simulink model "DEMOIO"  (Simulink 7.0)
settings: Solver=FixedStepDiscrete  StartTime=0.0  StopTime=10  FixedStep=0.0001  RelTol=1e-3
undefined symbols (not defined in the file or in its folder): OC1max
libraries: dsPICdrivers x4
CloseFcn:
  | rtwprivate ssgencode ModelCloseRequest speed_current_control
settings Model: Creator=Lubin  LastModifiedBy=MATLABMICROCHIP
settings SolverCC: PositivePriorityOrder=on  AutoInsertRateTranBlk=on
settings DataIOCC: Decimation=4  MaxDataPoints=65536
settings OptimizationCC: OptimizeModelRefInitCode=on  LifeSpan=1
settings DebuggingCC: SaveWithParameterizedLinksMsg=none  SignalResolutionControl=TryResolveAllWithWarning
settings HardwareCC: ProdBitPerInt=16  ProdEndianess=LittleEndian  ProdWordSize=16  ProdHWDeviceType=16-bit Generic  TargetHWDeviceType=32-bit Generic
settings RTWCC: SystemTargetFile=dspic.tlc  TemplateMakefile=dspic_pic30_gcc.tmf  PostCodeGenCommand=dsPIC_Compile()  Description=Embedded Target for Microchip dsPIC (real-time)  ProcessScript=dspic_make_rtw_hook
settings CodeAppCC: IgnoreCustomStorageClasses=off
settings STFCustomTargetCC: GenFloatMathFcnCalls=ANSI_C  ModelReferenceCompliant=off  IncludeMdlTerminateFcn=off  CombineOutputUpdateFcns=on  SuppressErrorStatus=on  ERTCustomFileBanners=on  SupportContinuousTime=off  SupportNonInlinedSFcns=off  SystemTargetFile=dspic.tlc
settings ERTTargetCC: GenFloatMathFcnCalls=ANSI_C  ModelReferenceCompliant=off  CompOptLevelCompliant=off  IncludeMdlTerminateFcn=off  SuppressErrorStatus=on  ModelStepFunctionPrototypeControlCompliant=off  InlinedParameterPlacement=NonHierarchical  ERTSrcFileBannerTemplate=dsPIC_code_template.cgt  ERTHdrFileBannerTemplate=dsPIC_code_template.cgt  ERTDataSrcFileTemplate=dsPIC_code_template.cgt  ERTDataHdrFileTemplate=dsPIC_code_template.cgt  ERTCustomFileTemplate=dsPIC_main.tlc
settings CustomProperty: DataType=string  Value=C:\MATLAB~4\bin\win32\gmake

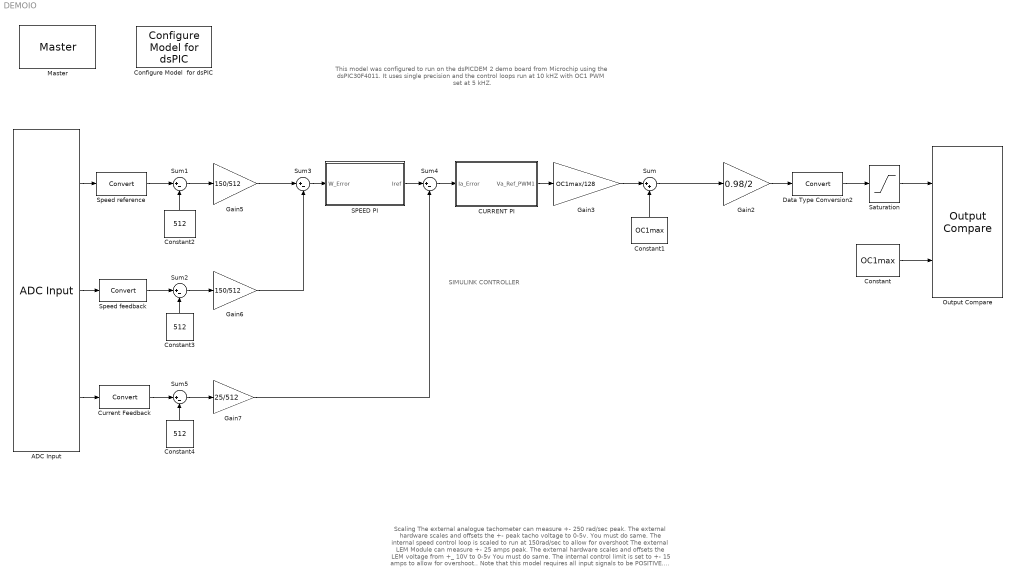
== system DEMOIO ==
  note: This model was configured to run on the dsPICDEM 2
      | demo board from Microchip using the  dsPIC30F4011.
      |
      | It uses single precision and the control loops run at 10 kHZ
      | with OC1 PWM set at  5 kHZ.
  note: Scaling
      |
      | The external analogue tachometer can measure +- 250 rad/sec peak. The external hardware scales and offsets the +- peak tacho voltage to  0-5v. You must do same. The internal speed control loop is scaled to run at 150rad/sec to allow for overshoot
      |
      | The external LEM Module can measure +- 25 amps peak. The external hardware scales and offsets the LEM voltage from +_ 10V to 0-5v You must do same. The internal control limit is set to +- 15 amps to allow for overshoot..
      |
      | Note that this model requires all input signals to be POSITIVE. The DC voltage is 128 volts. Change this to your desired output DC voltage.
      |
      | GOOD LUCK IT SHOULD WORK IF ALL THE FEEDBACK IS CORRECT.
      |
      | If you remove just the SIMULINK CNTROLLER you will be able to use the controllers in SIMULINK.
  note: SIMULINK CONTROLLER
  ADC Input : dsPICdrivers/Peripheral I//O/ADC Input  Tag=dsPIC_ADC  Priority=5  ADC_TYPE=10 bits  ADC_MODE=Continuous sampling & get last channel value  NbrSampleStep=1  VoltRefpopup="AVdd  -  AVss"  OutFormatBitspopup=0000 00dd dddd dddd : Integer  InterruptPriority=6  ANCHANNELS=[4 6 7]  MaxName=ANmax = 1024  Rin=1e2  ADCS=4  SAMC=1  Temperature=25  DMAChannel=0  SampleTime=0.0001  Status="OK  |  Tsmp=1.695e-007 |  T/Channel=2.204e-006 |  Tall=6.612e-006"
  CURRENT PI : Subsystem
  Configure Model  for dsPIC : dsPICdrivers/Simulink Configuration/Configure Model  for dsPIC
  Constant : Constant  Value=OC1max  OutDataTypeMode=uint16  OutDataType=sfix(16)  OutScaling=2^0  SampleTime=0.0001
  Constant1 : Constant  Orientation=up  Value=OC1max  OutDataTypeMode=single  OutDataType=sfix(16)  OutScaling=2^0  SampleTime=0.0001
  Constant2 : Constant  Orientation=up  Value=512  VectorParams1D=off  OutDataTypeMode=single  OutDataType=sfix(16)  OutScaling=2^0  SampleTime=0.0001
  Constant3 : Constant  Orientation=up  Value=512  OutDataTypeMode=single  OutDataType=sfix(16)  OutScaling=2^0  SampleTime=0.0001
  Constant4 : Constant  Orientation=up  Value=512  OutDataTypeMode=single  OutDataType=sfix(16)  OutScaling=2^0  SampleTime=0.0001
  Current Feedback : DataTypeConversion  OutDataTypeMode=single  OutDataType=sfix(16)  OutScaling=2^0  SampleTime=0.0001
  Data Type Conversion2 : DataTypeConversion  OutDataTypeMode=uint16  OutDataType=sfix(16)  OutScaling=2^0  SampleTime=0.0001
  Gain2 : Gain  Gain=0.98/2  ParameterDataType=sfix(16)  ParameterScaling=2^0  OutDataTypeMode=single  OutDataType=sfix(16)  OutScaling=2^0  SampleTime=0.0001
  Gain3 : Gain  Gain=OC1max/128  ParameterDataType=sfix(16)  ParameterScaling=2^0  OutDataTypeMode=single  OutDataType=sfix(16)  OutScaling=2^0  SampleTime=0.0001
  Gain5 : Gain  Gain=150/512  ParameterDataType=sfix(16)  ParameterScaling=2^0  OutDataType=sfix(16)  OutScaling=2^0  SampleTime=0.0001
  Gain6 : Gain  Gain=150/512  ParameterDataType=sfix(16)  ParameterScaling=2^0  OutDataType=sfix(16)  OutScaling=2^0  SampleTime=0.0001
  Gain7 : Gain  Gain=25/512  ParameterDataType=sfix(16)  ParameterScaling=2^0  OutDataType=sfix(16)  OutScaling=2^0  SampleTime=0.0001
  Master : dsPICdrivers/Master  Tag=dsPIC_MASTER  Priority=1  TimeStepType=Timer1  picType=30f4011  fcy=14745600  Quartz_33f=5e6  PLLActive_33f=off  fcyDesired_33f=0  tmr1="[1  1474  -0.029839]"  tmr1Info="Time Step : 0.00010003  ;   Error : -0.029839%  PR1=1474"  tmr2345="[1  0  0  0]"  tmr2345cfg=[-1 -1 -1 -1]  IOautoConf=on  typePort="[ 0  0  0  0  0  0  0  0  0  0  0  0  0  0  0  0  0  0  0  0  8  0  8  8  0  0  0  0  0  0  0  0  0  0  0  0  0  0  0  0  0  0  0  0  0  0  0  0  7  0  0  0  0  0  0  0  0  0  0  0  0  0  0  0  0  0  0  0  0  0  0  0  0  0  0  0  0  0  0  0  0  0  0  0  0  0  0  0  0  0  0  0  0  0  0  0  0  0  0  0  0  0  0  0  0  0  0  0  0  0  0  0 ]"  TRIS="[ 65535  65535  65535  65534  65535  65535  65535 ]"  ADPCFG=0  MasterBusyPort=None  MasterOverloadPort=None  FOSC=XT_PLL8  ClockSwitchMonitor=Both disabled  TempProtection_33f=TEMP_ON  FPBOR=PBOR_OFF  PWRT=PWRT_OFF  MCLR=MCLR_DIS  PowerSave=off  OverrideFcy=off  NewFcy=1e6
  Output Compare : dsPICdrivers/Peripheral I//O/Output Compare  Tag=dsPIC_PWM_out  Priority=5  IntPriority=3  CHANNEL=[1]  Channel_UP_Down_Periode=[5]  MaxChannel=[0.0002]  MaxName=' OC1max '  Precision=[11.5261]  Timer=[2]  Status=OK  SafeMarge=[0]  PortLetter=[68]  PortNumber=[0]  MaxValues=[2949.12]
  SPEED PI : Subsystem
  Saturation : Saturate  UpperLimit=OC1max  LowerLimit=0
  Speed feedback : DataTypeConversion  OutDataTypeMode=single  OutDataType=sfix(16)  OutScaling=2^0  SampleTime=0.0001
  Speed reference : DataTypeConversion  OutDataTypeMode=single  OutDataType=sfix(16)  OutScaling=2^0  SampleTime=0.0001
  Sum : Sum  Inputs=|++  OutDataTypeMode=single  OutDataType=sfix(16)  OutScaling=2^0
  Sum1 : Sum  Inputs=|+-  OutDataTypeMode=single  OutDataType=sfix(16)  OutScaling=2^0  InputSameDT=on
  Sum2 : Sum  Inputs=|+-  OutDataTypeMode=single  OutDataType=sfix(16)  OutScaling=2^0  InputSameDT=on
  Sum3 : Sum  Inputs=|+-  OutDataType=sfix(16)  OutScaling=2^0
  Sum4 : Sum  Inputs=|+-  OutDataType=sfix(16)  OutScaling=2^0
  Sum5 : Sum  Inputs=|+-  OutDataTypeMode=single  OutDataType=sfix(16)  OutScaling=2^0  InputSameDT=on
  wires:
  Constant/1 -> Output Compare/2
  Sum/1 -> Gain2/1
  ADC Input/1 -> Speed reference/1
  Constant2/1 -> Sum1/2
  ADC Input/2 -> Speed feedback/1
  Constant3/1 -> Sum2/2
  Sum1/1 -> Gain5/1
  Sum2/1 -> Gain6/1
  Gain2/1 -> Data Type Conversion2/1
  Data Type Conversion2/1 -> Saturation/1
  Sum3/1 -> SPEED PI/1(W_Error)
  CURRENT PI/1(Va_Ref_PWM1) -> Gain3/1
  Gain3/1 -> Sum/1
  Constant1/1 -> Sum/2
  Speed feedback/1 -> Sum2/1
  Saturation/1 -> Output Compare/1
  Sum4/1 -> CURRENT PI/1(Ia_Error)
  Constant4/1 -> Sum5/2
  Sum5/1 -> Gain7/1
  Current Feedback/1 -> Sum5/1
  ADC Input/3 -> Current Feedback/1
  Gain7/1 -> Sum4/2
  Speed reference/1 -> Sum1/1
  Gain5/1 -> Sum3/1
  SPEED PI/1(Iref) -> Sum4/1
  Gain6/1 -> Sum3/2

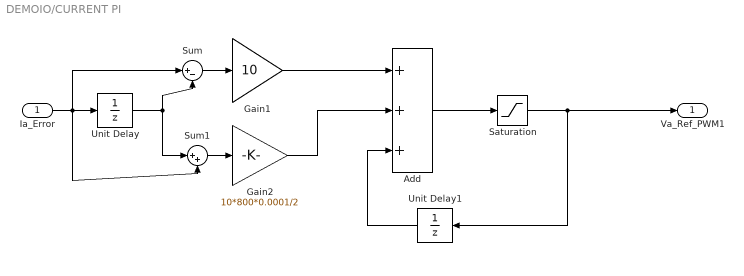
== system DEMOIO/CURRENT PI ==
  Ia_Error : Inport  OutDataType=sfix(16)  OutScaling=2^0
  Add : Sum  Inputs=+++  OutDataType=sfix(16)  OutScaling=2^-10
  Gain1 : Gain  Gain=10  ParameterDataType=sfix(16)  ParameterScaling=2^0  OutDataType=sfix(16)  OutScaling=2^0
  Gain2 : Gain  Gain=10*800*0.0001/2  ParameterDataType=sfix(16)  ParameterScaling=2^0  OutDataType=sfix(16)  OutScaling=2^0
  Saturation : Saturate  UpperLimit=128  LowerLimit=-128
  Sum : Sum  Inputs=|+-  OutDataType=sfix(16)  OutScaling=2^0
  Sum1 : Sum  Inputs=|++  OutDataType=sfix(16)  OutScaling=2^0
  Unit Delay : UnitDelay  SampleTime=1/5000
  Unit Delay1 : UnitDelay  Orientation=left  SampleTime=1/5000
  Va_Ref_PWM1 : Outport  OutDataType=sfix(16)  OutScaling=2^0
  wires:
  Ia_Error/1 -> Unit Delay/1, Sum/1, Sum1/2
  Unit Delay/1 -> Sum/2, Sum1/1
  Sum/1 -> Gain1/1
  Sum1/1 -> Gain2/1
  Gain1/1 -> Add/1
  Gain2/1 -> Add/2
  Add/1 -> Saturation/1
  Unit Delay1/1 -> Add/3
  Saturation/1 -> Unit Delay1/1, Va_Ref_PWM1/1

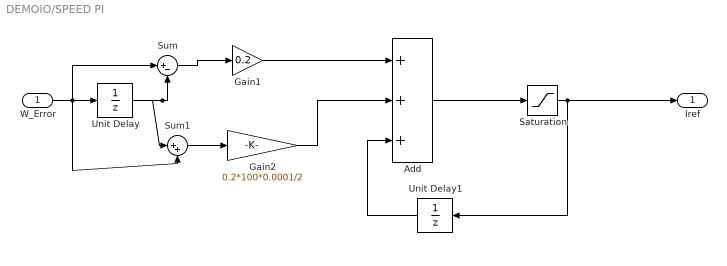
== system DEMOIO/SPEED PI ==
  W_Error : Inport  OutDataType=sfix(16)  OutScaling=2^0
  Add : Sum  Inputs=+++  OutDataType=sfix(16)  OutScaling=2^-10
  Gain1 : Gain  Gain=0.2  ParameterDataType=sfix(16)  ParameterScaling=2^0  OutDataType=sfix(16)  OutScaling=2^0
  Gain2 : Gain  Gain=0.2*100*0.0001/2  ParameterDataType=sfix(16)  ParameterScaling=2^0  OutDataType=sfix(16)  OutScaling=2^0
  Saturation : Saturate  UpperLimit=15  LowerLimit=-15
  Sum : Sum  Inputs=|+-  OutDataType=sfix(16)  OutScaling=2^0
  Sum1 : Sum  Inputs=|++  OutDataType=sfix(16)  OutScaling=2^0
  Unit Delay : UnitDelay  SampleTime=1/5000
  Unit Delay1 : UnitDelay  Orientation=left  SampleTime=1/5000
  Iref : Outport  OutDataType=sfix(16)  OutScaling=2^0
  wires:
  Saturation/1 -> Unit Delay1/1, Iref/1
  Unit Delay1/1 -> Add/3
  Add/1 -> Saturation/1
  Gain2/1 -> Add/2
  Gain1/1 -> Add/1
  Sum1/1 -> Gain2/1
  Sum/1 -> Gain1/1
  Unit Delay/1 -> Sum1/1, Sum/2
  W_Error/1 -> Sum1/2, Sum/1, Unit Delay/1
